simulink model "Sample_task"  (Simulink 8.1)
settings: Solver=ode4  SolverMode=SingleTasking  StartTime=0.0  StopTime=inf  FixedStep=0.0005  RelTol=1e-3
model workspace (MAT data in the model file):
  BKIN_STEP_TIME = 0.0005
  col_x = 1
  col_y = 2
  WIDTH = 3
  HEIGHT = 4
  TARGET_COL = 1
  LOAD = 2
  TRAJ_DURATION_COL = 3
  MAX_LOAD = 2
  FORCE_ON = 1
  HAND_RADIUS = 6
  REST_COL = 4
  TRAINING_COL = 5
  HAND_COLOR = 5
  TARGET_STROKE = 8
  TARGET_RADIUS = 9
  xMaxCursor = 15
  yMaxCursor = 16
  TARGET_COLOR = 7
  START_X = 10
  START_Y = 11
  END_X = 12
  END_Y = 13
  OPACITY_GRADIENT : num (value not decoded)
StartFcn:
  |  warndlg('Dexterit-E models cannot run under simulation. Please compile your model and run it from within Dexterit-E.');set_param(bdroot,'SimulationCommand','stop')
undefined symbols (not defined in the file or in its folder): slselsubs
libraries: simulink x4, General x3, KINARM_loads x2, KINARM_IO x1, KINARM_EP_loads x1, Video x1, xpclib x1
(part 1 of 3)
CloseFcn:
  | rtwprivate ssgencode ModelCloseRequest b2lab2d
settings Model: Creator=Chris Grebeldinger  LastModifiedBy=BKIN TECHNOLOGIES  ModifiedComment=chris -- Wed Feb 16 09:18:30 2005 -- Version 1.1384  ModifiedHistory=Feb 16/05 - Add error repeat, add offset ramp  ExtModeArmWhenConnect=off  ExtModeLogAll=off  BufferReuse=off
settings DataIOCC: LimitDataPoints=off  SaveOutput=off  SaveTime=off  SignalLoggingName=sigsOut
settings OptimizationCC: BlockReduction=off  BooleanDataType=off  OptimizeBlockIOStorage=off  BufferReuse=off  ExpressionFolding=off  FoldNonRolledExpr=off  LocalBlockOutputs=off  InitFltsAndDblsToZero=on
settings DebuggingCC: SaveWithParameterizedLinksMsg=none  SignalResolutionControl=TryResolveAllWithWarning  SolverPrmCheckMsg=none  MultiTaskDSMMsg=warning  MultiTaskCondExecSysMsg=none  StrictBusMsg=None
settings HardwareCC: ProdIntDivRoundTo=Zero  ProdEndianess=LittleEndian  ProdHWDeviceType=Generic->32-bit x86 compatible  TargetHWDeviceType=32-bit Generic
settings SFSimCC: SimParseCustomCode=off
settings RTWCC: SystemTargetFile=xpctarget.tlc  TemplateMakefile=xpc_default_tmf  Description=xPC Target  ProcessScript=xpctarget_make_rtw_hook  IncludeERTFirstTime=on  RTWCompilerOptimization=On
settings CodeAppCC: MaxIdLength=63
settings xpcTargetCC: TargetFcnLib=ansi_tfl_tmw.mat  CodeReplacementLibrary=XPC_BLAS  ParMdlRefBuildCompliant=on  ConcurrentExecutionCompliant=on  CombineSignalStateStructs=off  MATLABClassNameForMDSCustomization=xpcAperiodicCustomization  GRTInterface=on  GenerateAllocFcn=off  xPCTaskExecutionProfile=off  xPCRL32EventNumber=5000  xPCisDownloadable=off  xPCLoadParamSetFile=off  xPCConcurrentTasks=off  xPCEnableSFAnimation=off

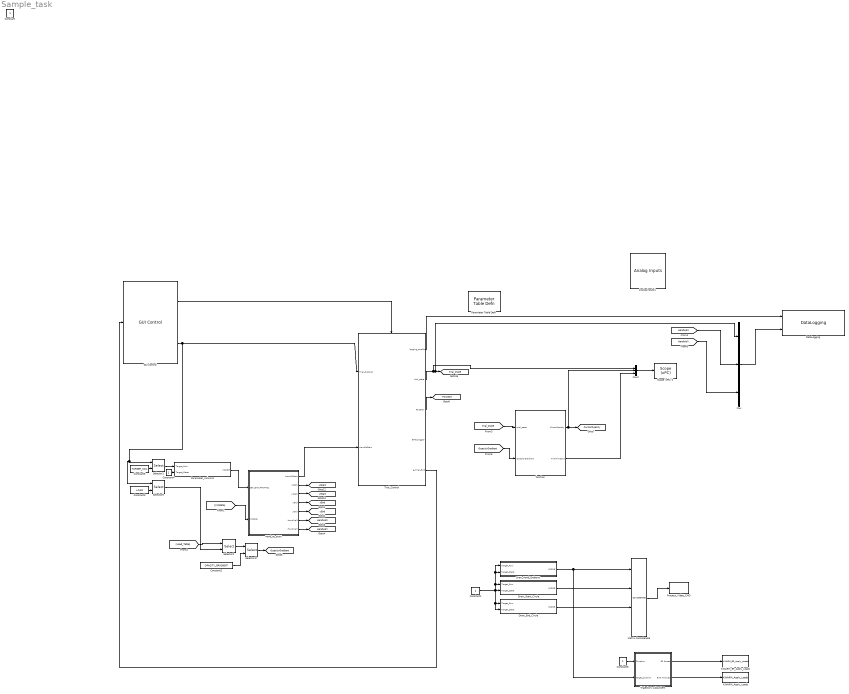
== system Sample_task ==
  Analog Inputs1 : KINARM_IO/Analog Inputs  channel=[5,6,7,8,9,10]  range=[5]  coupling=[0]  scantime6071e=1.28e-5  scantime6229=5e-6  sampletime=0.001  slot=-1  oscantime6071e=0
  Constant1 : Constant
  Constant2 : Constant  Value=OPACITY_GRADIENT
  Constant3 : Constant  Value=LOAD
  Constant4 : Constant
  Constant5 : Constant  Value=TARGET_COL
  Constant6 : Constant
  DataLogging : General/DataLogging  log_event_codes=off  log_analog_inputs=on
      link override Poll KINARM/EPTorqueCMD: GotoTag=KINARMEPTorqueCMD
      link override Poll KINARM/TorqueCMD: GotoTag=KINARMTorqueCMD
      link override Poll KINARM/ZeroEPTorque: Value=[0 0 0 0]
      link override Poll KINARM/ZeroTorque: Value=[0 0 0 0]
  Draw_End_Circle : Subsystem  AncestorBlock=Video/Show_Target_With_Label  mask(Show_Target_With_Label){target_type=Circle, num_states=1, attribcol1=[TARGET_COLOR TARGET_COLOR TARGET_STROKE TARGET_RADIUS 0 0 0], attribcol2=[6 6 0 3 0 0 0], attribcol3=[0 0 0 0 0 0 0], attribcol4=[0 0 0 0 0 0 0], attribcol5=[0 0 24 0 0 0 0], stateindices_padding=[0 0 0 0;0 0 0 0;0 0 0 0;0 0 0 0;0 0 0 0], source=dialog, opacity=100, target_display=Both subject and operator displays}
      mask prompts: target_type "Type of Target"; num_states "Number of Target States"; attribcol1 "State 1 Target Table Column(s)"; attribcol2 "State 2 Target Table Column(s)"; attribcol3 "State 3 Target Table Column(s)"; attribcol4 "State 4 Target Table Column(s)"; attribcol5 "State 5 Target Table Column(s)"; stateindices_padding "State Indices Padding"; source "Source for Opacity"; target_display "Target Display"
      mask help: This block returns a VCODE that, when sent to the Process_Video_CMD block, will cause a single target with a text label to be drawn. The label will be centered at the centroid of the target. Target parameters are specified in the Target Table according to the columns defined below and the row input to this block.
      mask init:
      | block_path = gcb;  % store block path, as gcb may change with block operations
      | 
      | %%% Get the model's workspace, because it is required to evaluate constants from the Parameter Table Def'n block
      | modelName=bdroot(block_path);
      | modelWorkspace = get_param(modelName, 'ModelWorkspace');
      | 
      | %%% Handle background colours if link status changes.  
      | checkBackgroundColour(block_path, 'Video');
      | 
      | %%% create the names of the input and output ports to display on the mask
      | output_block=char(find_system(block_path,'LookUnderMasks','all','FollowLinks','on','SearchDepth',1,'BlockType','Outport'));
      | outputname=get_param(output_block,'Name');
      | 
      | input_block=find_system(block_path,'LookUnderMasks','all','FollowLinks','on','SearchDepth',1,'BlockType','Inport');
      | inputname1=get_param(char(input_block{1}),'Name');
      | inputname2=get_param(char(input_block{2}),'Name');
      | if length(input_block) >= 3
      |     inputname3=get_param(char(input_block{3}),'Name');
      | end
      | 
      | %%%%%%%%%%%%%%%%%%%%%%%%%%%%%%%%%%%%%%%%%%%%%%%%%%%%%%%%%%%%%
      | %%% Create or replace the opacity input port
      | % Note: in earlier versions of MATLAB, the replace_block function did not work properly. When we drop support for R2007b,
      | % Check to see if it works properly in R2010a and if so, then this code can be simplified with the use of the replace_block function
      | sourceStr=get_param(block_path,'source');
      | 
      | if strmatch(sourceStr, 'dialog')
      | 	if length(input_block) == 3
      | 		pos=get_param([block_path '/Opacity'],'position');
      | 		delete_line(block_path, 'Opacity/1', 'Embedded MATLAB Function/4');
      | 		delete_block(input_block{3});
      |         add_block('built-in/Constant',[block_path '/Opacity'],'Name','Opacity');
      | 		set_param([block_path '/Opacity'],'position',pos);
      | 		add_line(block_path, 'Opacity/1', 'Embedded MATLAB Function/4');
      | 		set_param([block_path '/Opacity'],'Value','opacity');
      | 	end
      | 	displaytext = ['disp(columntext); port_label(''output'',1,outputname); port_label(''input'',1, inputname1); port_label(''input'',2, inputname2);'];
      | else
      | 	if length(input_block) == 2
      | 		pos=get_param([block_path '/Opacity'],'position');
      | 		delete_line(block_path, 'Opacity/1', 'Embedded MATLAB Function/4');
      | 		delete_block([block_path, '/Opacity']);
      | 		add_block('built-in/Inport',[block_path '/In2'],'Name','Opacity');
      | 		set_param([block_path '/Opacity'],'position',pos);
      | 		add_line(block_path, 'Opacity/1', 'Embedded MATLAB Function/4');
      |  	end
      | 	inputname3='Opacity';
      | 	displaytext = ['disp(columntext); port_label(''output'',1,outputname); port_label(''input'',1, inputname1); port_label(''input'',2, inputname2); port_label(''input'',3, inputname3);'];
      | end
      | set_param(block_path,'MaskDisplay',displaytext);
      | 
      | 
      | %%%%%%%%%%%%%%%%%%%%%%%%%%%%%%%%%%%%%%%%%%%%%%%%%%%%%%%%%%%%%
      | %%% Check and format the input strings for the vectors of column entires
      | targetTypeStr=get_param(block_path, 'target_type');
      | 
      | switch targetTypeStr(1:3)
      | 	case 'Cir',		numCol = 7;
      | 	case 'Ell',		numCol = 9;
      |     case 'Rec',		numCol = 9;
      |     case 'Lin',		numCol = 8;
      |     case 'Tri',		numCol = 10;
      | 	otherwise,		numCol = 7;
      | end
      | 
      | % % % numCol=str2num( get_param(block_path, 'num_col') );
      | for ii = 1:5
      | 	variableName = ['attribcol' num2str(ii)];
      | 	attribcoltext = get_param(block_path, variableName);
      | 	attribcoltext = checkUserInputVectorLength(attribcoltext, numCol);
      | 	set_param(block_path, variableName, attribcoltext);
      | end
      | 
      | % the input to the Embedded MATLAB script under the mask needs to have a certain size. This creates 'padding' to add to the 
      | % attribcol vectors to get to that size
      | zeros_5x7_matrix = zeros(5,7);
      | set_param(block_path, 'stateindices_padding', mat2str(zeros_5x7_matrix(:, 1:(11-numCol))) );
      | 
      | 
      | %%%%%%%%%%%%%%%%%%%%%%%%%%%%%%%%%%%%%%%%%%%%%%%%%%%%%%%%%%%%%
      | %%% Create the text to show on the mask
      | numStates = str2num(get_param(block_path, 'num_states'));
      | 
      | for ii = 1:numStates
      | 	variableName = ['attribcol' num2str(ii)];
      | 	attribcolString = get_param(block_path, variableName);
      | 	if isempty(modelWorkspace)
      | 		% if the block is part of a library, then modelWorkspace will be empty and the other code to evaluate attribcolStringEval will fail
      | 		attribcolStringEval = '[4 0 3 0 0 0 0]';
      | 	else
      | 		[attribcolValue, errorMessage] = BKINevalin(modelWorkspace, attribcolString);
      | 		attribcolStringEval = ['          ' mat2str( attribcolValue )];
      | 	end
      | 	if ii > 1
      | 		columntext = strvcat(columntext, attribcolStringEval);
      | 	else
      | 		columntext = attribcolStringEval;
      | 	end
      | end
      | 
      | % Add formatting spaces so that the mask looks nice
      | space = repmat(' ', 1, round(length(columntext)/2));
      | columntext=strvcat([space '(columns)'], columntext);
      mask Help:
      | Used to draw a single, stationary target with a label.
      | 
      | <H2>Library </H2>
      | Video
      | 
      | <H2>Description </H2>
      | This block returns a VCODE, which when sent to the Process_Video_CMD block will draw a single stationary target with a label. The VCODE contains all of the target parameters necessary to draw the target and the label.
      | <P>
      | The VCODE is generated from information contained in the Target Table. Which parts of the Target Table are used is determined by the columns selected (see Parameters and Dialog Box below).<P>
      | 
      | <p>For example, assume the "row" input is 2, the "type of target" is set to "rectangle" and the "Target Table Columns" is set to [3 0 0 4 5 0 6 7 4].
      | Then using the sample target table below a red rectangle will be drawn at (20cm, 40cm) with a width of 10cm and a height of 3cm.
      | The rectangle will have the word "Maybe" in yellow on it in letters 3cm heigh. The zeros in the  "Target Table Columns" indicate those parameters are not used (i.e. no stroke color, no stroke width, and no rotation).
      | 
      | <p><tt>
      | ______________________________________________________________________<br>
      | |&nbsp;&nbsp;&nbsp;&nbsp;&nbsp;&nbsp;&nbsp;&nbsp;&nbsp;&nbsp;| X Pos | Y pos |&nbsp;&nbsp;Fill | Width | Height |&nbsp;&nbsp;Text | TColor |<br>
      | ----------------------------------------------------------------------<br>
      | | target 1 |&nbsp;&nbsp;&nbsp;&nbsp;10 |&nbsp;&nbsp;&nbsp;&nbsp;10 | white |&nbsp;&nbsp;&nbsp;&nbsp;&nbsp;5 |&nbsp;&nbsp;&nbsp;&nbsp;&nbsp;&nbsp;2 |&nbsp;&nbsp;&nbsp;Yes |&nbsp;&nbsp;green |<br>
      | | target 2 |&nbsp;&nbsp;&nbsp;&nbsp;20 |&nbsp;&nbsp;&nbsp;&nbsp;40 |&nbsp;&nbsp;&nbsp;red |&nbsp;&nbsp;&nbsp;&nbsp;10 |&nbsp;&nbsp;&nbsp;&nbsp;&nbsp;&nbsp;3 | Maybe | yellow |<br>
      | | target 3 |&nbsp;&nbsp;&nbsp;-40 |&nbsp;&nbsp;&nbsp;&nbsp;10 |&nbsp;&nbsp;blue |&nbsp;&nbsp;&nbsp;&nbsp;&nbsp;3 |&nbsp;&nbsp;&nbsp;&nbsp;&nbsp;&nbsp;4 | Wrong |&nbsp;&nbsp;&nbsp;&nbsp;red |
      | ----------------------------------------------------------------------<br>
      | 
      | 
      | </tt>
      | 
      | 
      | <p>Inputs:<br>
      | <B> Target_Row: </B> this scalar input determines which row in the Target Table is used to define the target parameters. Typically the Target_Row comes from the Trial_Protocol.  <P>
      | <B> Target_State: </B> this scalar input determines which state the target is in. Different states reference different columns in the Target Table (as defined in the Dialog Box). Typically the Target_State input is controlled by the Stateflow chart to dynamically change the appearance of the target depending on system and/or subject behavior. Target_State=0 is a valid input, which turns the target off. The intended method for turning a target off is to set Target_State=0. <BR>
      | <P>
      | <B>Opacity:</B> This input is only available if Source for Opacity is selected as port, in which case the opacity for all of the targets created by this block is specified as a percentage.
      | The length of this input must either match the length of the Target_Row(s) input (i.e. which case each Opacity maps to the appropriate Target_row)
      | or this input must be a scalar (in which case the Opacity maps to all of the Target_Rows).<BR>
      | <P>
      | There is one output from this block:
      | <P>
      | <B> VCODE: </B> this output is a vector containing one VCODE. This output must go to the Process_Video_CMD block of the video library for the target to actually be shown (if any other visual targets are to be displayed, then this VCODE output must be concatenated with the other VCODES prior to connection to the Process_Video_CMD block - see Help for the Process_Video_CMD block for more information).
      | <P>
      | To show multiple targets simultaneously, multiple copies of the Show_Target and Show_Target_With_Label blocks can be used in a Task Program. The output VCODES from multiple Show_Target and Show_Target_With_Label blocks must be concatenated prior to connection to the Process_Video_CMD block.
      | <P>
      | 
      | <H2>Parameters and Dialog Box</H2>
      | <B>Type of Target:</B> Choose the type of target specified in the target table.
      | <P>
      | <B>Number of Target States:</B> Choose the number of target states specified in each target row. Up to five target states are allowed per target row.
      | <P>
      | <B>State [n] Target Table Columns:</B> Enter the column indices that specify the relevant target attributes in the Target Table. All target types have the same first three target attributes (fill colour, stroke colour and stroke width) and the same last three target attributes (label text, label colour, and label height).
      | <Blockquote>
      | <P>
      | Element 1 (fill colour) - points to the column index in the Target Table containing the fill colour. If this index is 0, then the fill colour is transparent and the Target Table is not referenced. For line targets, the fill colour is not used.
      | <P>
      | Element 2 (stroke colour) - points to the column index in the Target Table containing the stroke colour. If this index is 0, then the stroke colour is transparent and the Target Table is not referenced. It is possible to use the same column index for both fill colour and stroke colour (i.e.  if single-colour targets are desired). For line targets, stroke colour defines the colour of the line.
      | <P>
      | Element 3 (stroke width) - points to the column index in the Target Table containing the stroke width (cm). If no stroke is desired, then setting the stroke column index to 0 will produce a stroke width of 0  and the Target Table is not referenced.  Setting stroke column index to a value less than 0 will produce a standard 1 mm stroke width, again without referencing the Target Table. For line targets, stroke width defines the width of the line.
      | <P>
      | <B><I>Circle</I></B> <P>
      | Element 4 (radius) - radius of the circle (cm).
      | <P>
      | <B><I>Ellipse</I></B> <P>
      | Elements 4-6 (ellipse properties) - major radius (cm), minor radius (cm), rotation angle (degrees). If no rotation is desired, then setting rotation column index to 0 will produce a default rotation of 0 and the Target Table will not be referenced.
      | <P>
      | <B><I>Rectangle</I></B><P>
      | Elements 4-6 (rectangle properties) - length (cm), height (cm), rotation angle (degrees). If no rotation is desired, then setting rotation column index to 0 will produce a default rotation of 0 and the Target Table will not be referenced.
      | <P>
      | <B><I>Line</I></B><P>
      | Elements 4-5 (line properties) - end point x-axis position relative to start point (cm), end point y-axis position relative to start point (cm). The width and colour of the line are defined by the stroke width and the stroke colour, respectively. The fill colour column is ignored (i.e. any value can be used for column 1)
      | <P>
      | <B><I>Triangle</I></B><P>
      | Elements 4-7 (triangle properties) - length (cm), height (cm), offset of peak of triangle relative to midpoint of the length (cm), rotation angle (degrees). If a height column index of 0 is specified, then an equilateral triangle with sides of the specified length will be created and the Target Table will not be referenced for height or peak offset. If no rotation is desired, then setting a rotation column index of 0 will produce a default rotation of 0 and the Target Table will not be referenced.
      | <P>
      | <B><I>Label</I></B>
      | <P>
      | The last three elements of the target state vector define the label. In order, these elements are:
      | <P>
      | Label text - the index of the column in the Target Table containing the text used for the label (up to 50 characters).
      | <P>
      | Label colour - the index of the column in the Target Table containing the label colour. If this index is 0, then the label colour is transparent and the Target Table is not referenced.
      | <P>
      | Label height - the index of the column in the Target Table containing the label height (cm).
      | </Blockquote>
      | <P>
      | Each target state requires its own set of column index definitions (although multiple states can point to the same column index if desired).<P>
      | 
      | <B>Source for Opacity:</B> Choose either dialog, to specify the opacity in this dialog, or port, which will create a new input to allow dynamic control of opacity.
      | <P>
      | <B>Opacity:</B> This parameter is only available if Source for Opacity is selected as dialog, in which case the opacity for all of the targets created by this block is specified as a percentage.
      | <P>
      | <B>Target Display:</B> This option determines whether the target(s) are shown on the operator display only, the subject display only, or both displays.
      | <P>
      | 
      | <H2>Examples</H2>
      | 
      | <B>Example 1:</B>  Suppose a target row will be used to define 1 state for an ellipse type target. It will be an outline of an ellipse with a label in the center (using a stroke colour and a standard 1mm stroke width). The related Target Table columns are:
      | <P>
      | column 4 = colour<BR>
      | column 5 = major radius<BR>
      | column 6 = minor radius<BR>
      | column 7 = orientation<BR>
      | column 8 = label text<BR>
      | column 9 = label colour<BR>
      | column 10 = label height
      | <P>For this example, "State 1 Target Table Columns" would equal [0 4 -1 5 6 7 8 9 10].
      | <P>
      | 
      | <H2>Related Blocks </H2>
      | Show_Target<BR>
      | Process_Video_CMD
      mask TypeOptions target_type: Circle | Ellipse | Rectangle | Line | Triangle
      mask Callback target_type:
      | %%%%
      | % Because of bugs iN R2007, R2010a and R2013a (which have been reported to Mathworks), the following code
      | % is required here because in the Initialization Section it will ONLY correctly update those Mask Parameters that are hidden
      | % when the OK button is clicked (NOTE: the initialization code will correctly update all Mask Parameters when the Apply button
      | % is clicked, the bug is that it should also update everything when the OK button is clicked in the absence of an Apply click)
      | %
      | % Adding a set_param call which updates one of the mask parameters will call the initialization code to run, which "avoids"
      | % this bug. This code should be removed once Mathworks has fixed this bug.
      | 
      | temp = get_param(gcb, 'target_type');
      | set_param(gcb, 'target_type', temp);
      mask TypeOptions num_states: 1 | 2 | 3 | 4 | 5
      mask Callback num_states:
      | block_path=gcb;
      | num_states=str2num(get_param(block_path, 'num_states'));
      | vis=get_param(block_path,'MaskVisibilities');
      | 
      | %If the number of states>1, then output an array instead of a vector.
      | %Only show those inputs necessary on the Mask
      | output_block=char(find_system(block_path,'LookUnderMasks','all','SearchDepth',1,'BlockType','Outport'));
      | if num_states==1			%output of HandInTarget block is a vector
      | 	vis{4}='off';
      | 	vis{5}='off';
      | 	vis{6}='off';
      | 	vis{7}='off';
      | elseif num_states==2					%output of HandInTarget block is an array
      | 	vis{4}='on';
      | 	vis{5}='off';
      | 	vis{6}='off';
      | 	vis{7}='off';
      | elseif num_states==3					%output of HandInTarget block is an array
      | 	vis{4}='on';
      | 	vis{5}='on';
      | 	vis{6}='off';
      | 	vis{7}='off';
      | elseif num_states==4					%output of HandInTarget block is an array
      | 	vis{4}='on';
      | 	vis{5}='on';
      | 	vis{6}='on';
      | 	vis{7}='off';
      | else								%output of HandInTarget block is an array
      | 	vis{4}='on';
      | 	vis{5}='on';
      | 	vis{6}='on';
      | 	vis{7}='on';
      | end
      | set_param(block_path,'MaskVisibilities',vis);
      mask TypeOptions source: dialog | port
      mask Callback source:
      | % Show or hide the opacity input on the mask dialog
      | sourceStr=get_param(gcb,'source');
      | vis=get_param(gcb,'MaskVisibilities');
      | 
      | if strmatch(sourceStr, 'dialog')
      | 	vis{10}='on';
      | else
      | 	vis{10}='off';
      | end
      | 
      | set_param(gcb,'MaskVisibilities',vis);
      mask TypeOptions target_display: Both subject and operator displays | Subject display only | Operator display only
      mask Display: disp(columntext); port_label('output',1,outputname); port_label('input',1, inputname1); port_label('input',2, inputname2);
  Draw_Hand_Endpoint : Subsystem  AncestorBlock=Video/Show_Target_With_Label  mask(Show_Target_With_Label){target_type=Circle, num_states=1, attribcol1=[HAND_COLOR 0 0 HAND_RADIUS 0 0 0], attribcol2=[6 6 0 3 0 0 0], attribcol3=[0 0 0 0 0 0 0], attribcol4=[0 0 0 0 0 0 0], attribcol5=[0 0 24 0 0 0 0], stateindices_padding=[0 0 0 0;0 0 0 0;0 0 0 0;0 0 0 0;0 0 0 0], source=dialog, opacity=100, target_display=Both subject and operator displays}
      mask prompts: target_type "Type of Target"; num_states "Number of Target States"; attribcol1 "State 1 Target Table Column(s)"; attribcol2 "State 2 Target Table Column(s)"; attribcol3 "State 3 Target Table Column(s)"; attribcol4 "State 4 Target Table Column(s)"; attribcol5 "State 5 Target Table Column(s)"; stateindices_padding "State Indices Padding"; source "Source for Opacity"; target_display "Target Display"
      mask help: This block returns a VCODE that, when sent to the Process_Video_CMD block, will cause a single target with a text label to be drawn. The label will be centered at the centroid of the target. Target parameters are specified in the Target Table according to the columns defined below and the row input to this block.
      mask init: same as Sample_task/Draw_End_Circle
      mask Help:
      | Used to draw a single, stationary target with a label.
      | 
      | <H2>Library </H2>
      | Video
      | 
      | <H2>Description </H2>
      | This block returns a VCODE, which when sent to the Process_Video_CMD block will draw a single stationary target with a label. The VCODE contains all of the target parameters necessary to draw the target and the label.
      | <P>
      | The VCODE is generated from information contained in the Target Table. Which parts of the Target Table are used is determined by the columns selected (see Parameters and Dialog Box below).<P>
      | 
      | <p>For example, assume the "row" input is 2, the "type of target" is set to "rectangle" and the "Target Table Columns" is set to [3 0 0 4 5 0 6 7 4].
      | Then using the sample target table below a red rectangle will be drawn at (20cm, 40cm) with a width of 10cm and a height of 3cm.
      | The rectangle will have the word "Maybe" in yellow on it in letters 3cm heigh. The zeros in the  "Target Table Columns" indicate those parameters are not used (i.e. no stroke color, no stroke width, and no rotation).
      | 
      | <p><tt>
      | ______________________________________________________________________<br>
      | |&nbsp;&nbsp;&nbsp;&nbsp;&nbsp;&nbsp;&nbsp;&nbsp;&nbsp;&nbsp;| X Pos | Y pos |&nbsp;&nbsp;Fill | Width | Height |&nbsp;&nbsp;Text | TColor |<br>
      | ----------------------------------------------------------------------<br>
      | | target 1 |&nbsp;&nbsp;&nbsp;&nbsp;10 |&nbsp;&nbsp;&nbsp;&nbsp;10 | white |&nbsp;&nbsp;&nbsp;&nbsp;&nbsp;5 |&nbsp;&nbsp;&nbsp;&nbsp;&nbsp;&nbsp;2 |&nbsp;&nbsp;&nbsp;Yes |&nbsp;&nbsp;green |<br>
      | | target 2 |&nbsp;&nbsp;&nbsp;&nbsp;20 |&nbsp;&nbsp;&nbsp;&nbsp;40 |&nbsp;&nbsp;&nbsp;red |&nbsp;&nbsp;&nbsp;&nbsp;10 |&nbsp;&nbsp;&nbsp;&nbsp;&nbsp;&nbsp;3 | Maybe | yellow |<br>
      | | target 3 |&nbsp;&nbsp;&nbsp;-40 |&nbsp;&nbsp;&nbsp;&nbsp;10 |&nbsp;&nbsp;blue |&nbsp;&nbsp;&nbsp;&nbsp;&nbsp;3 |&nbsp;&nbsp;&nbsp;&nbsp;&nbsp;&nbsp;4 | Wrong |&nbsp;&nbsp;&nbsp;&nbsp;red |
      | ----------------------------------------------------------------------<br>
      | 
      | 
      | </tt>
      | 
      | 
      | <p>Inputs:<br>
      | <B> Target_Row: </B> this scalar input determines which row in the Target Table is used to define the target parameters. Typically the Target_Row comes from the Trial_Protocol.  <P>
      | <B> Target_State: </B> this scalar input determines which state the target is in. Different states reference different columns in the Target Table (as defined in the Dialog Box). Typically the Target_State input is controlled by the Stateflow chart to dynamically change the appearance of the target depending on system and/or subject behavior. Target_State=0 is a valid input, which turns the target off. The intended method for turning a target off is to set Target_State=0. <BR>
      | <P>
      | <B>Opacity:</B> This input is only available if Source for Opacity is selected as port, in which case the opacity for all of the targets created by this block is specified as a percentage.
      | The length of this input must either match the length of the Target_Row(s) input (i.e. which case each Opacity maps to the appropriate Target_row)
      | or this input must be a scalar (in which case the Opacity maps to all of the Target_Rows).<BR>
      | <P>
      | There is one output from this block:
      | <P>
      | <B> VCODE: </B> this output is a vector containing one VCODE. This output must go to the Process_Video_CMD block of the video library for the target to actually be shown (if any other visual targets are to be displayed, then this VCODE output must be concatenated with the other VCODES prior to connection to the Process_Video_CMD block - see Help for the Process_Video_CMD block for more information).
      | <P>
      | To show multiple targets simultaneously, multiple copies of the Show_Target and Show_Target_With_Label blocks can be used in a Task Program. The output VCODES from multiple Show_Target and Show_Target_With_Label blocks must be concatenated prior to connection to the Process_Video_CMD block.
      | <P>
      | 
      | <H2>Parameters and Dialog Box</H2>
      | <B>Type of Target:</B> Choose the type of target specified in the target table.
      | <P>
      | <B>Number of Target States:</B> Choose the number of target states specified in each target row. Up to five target states are allowed per target row.
      | <P>
      | <B>State [n] Target Table Columns:</B> Enter the column indices that specify the relevant target attributes in the Target Table. All target types have the same first three target attributes (fill colour, stroke colour and stroke width) and the same last three target attributes (label text, label colour, and label height).
      | <Blockquote>
      | <P>
      | Element 1 (fill colour) - points to the column index in the Target Table containing the fill colour. If this index is 0, then the fill colour is transparent and the Target Table is not referenced. For line targets, the fill colour is not used.
      | <P>
      | Element 2 (stroke colour) - points to the column index in the Target Table containing the stroke colour. If this index is 0, then the stroke colour is transparent and the Target Table is not referenced. It is possible to use the same column index for both fill colour and stroke colour (i.e.  if single-colour targets are desired). For line targets, stroke colour defines the colour of the line.
      | <P>
      | Element 3 (stroke width) - points to the column index in the Target Table containing the stroke width (cm). If no stroke is desired, then setting the stroke column index to 0 will produce a stroke width of 0  and the Target Table is not referenced.  Setting stroke column index to a value less than 0 will produce a standard 1 mm stroke width, again without referencing the Target Table. For line targets, stroke width defines the width of the line.
      | <P>
      | <B><I>Circle</I></B> <P>
      | Element 4 (radius) - radius of the circle (cm).
      | <P>
      | <B><I>Ellipse</I></B> <P>
      | Elements 4-6 (ellipse properties) - major radius (cm), minor radius (cm), rotation angle (degrees). If no rotation is desired, then setting rotation column index to 0 will produce a default rotation of 0 and the Target Table will not be referenced.
      | <P>
      | <B><I>Rectangle</I></B><P>
      | Elements 4-6 (rectangle properties) - length (cm), height (cm), rotation angle (degrees). If no rotation is desired, then setting rotation column index to 0 will produce a default rotation of 0 and the Target Table will not be referenced.
      | <P>
      | <B><I>Line</I></B><P>
      | Elements 4-5 (line properties) - end point x-axis position relative to start point (cm), end point y-axis position relative to start point (cm). The width and colour of the line are defined by the stroke width and the stroke colour, respectively. The fill colour column is ignored (i.e. any value can be used for column 1)
      | <P>
      | <B><I>Triangle</I></B><P>
      | Elements 4-7 (triangle properties) - length (cm), height (cm), offset of peak of triangle relative to midpoint of the length (cm), rotation angle (degrees). If a height column index of 0 is specified, then an equilateral triangle with sides of the specified length will be created and the Target Table will not be referenced for height or peak offset. If no rotation is desired, then setting a rotation column index of 0 will produce a default rotation of 0 and the Target Table will not be referenced.
      | <P>
      | <B><I>Label</I></B>
      | <P>
      | The last three elements of the target state vector define the label. In order, these elements are:
      | <P>
      | Label text - the index of the column in the Target Table containing the text used for the label (up to 50 characters).
      | <P>
      | Label colour - the index of the column in the Target Table containing the label colour. If this index is 0, then the label colour is transparent and the Target Table is not referenced.
      | <P>
      | Label height - the index of the column in the Target Table containing the label height (cm).
      | </Blockquote>
      | <P>
      | Each target state requires its own set of column index definitions (although multiple states can point to the same column index if desired).<P>
      | 
      | <B>Source for Opacity:</B> Choose either dialog, to specify the opacity in this dialog, or port, which will create a new input to allow dynamic control of opacity.
      | <P>
      | <B>Opacity:</B> This parameter is only available if Source for Opacity is selected as dialog, in which case the opacity for all of the targets created by this block is specified as a percentage.
      | <P>
      | <B>Target Display:</B> This option determines whether the target(s) are shown on the operator display only, the subject display only, or both displays.
      | <P>
      | 
      | <H2>Examples</H2>
      | 
      | <B>Example 1:</B>  Suppose a target row will be used to define 1 state for an ellipse type target. It will be an outline of an ellipse with a label in the center (using a stroke colour and a standard 1mm stroke width). The related Target Table columns are:
      | <P>
      | column 4 = colour<BR>
      | column 5 = major radius<BR>
      | column 6 = minor radius<BR>
      | column 7 = orientation<BR>
      | column 8 = label text<BR>
      | column 9 = label colour<BR>
      | column 10 = label height
      | <P>For this example, "State 1 Target Table Columns" would equal [0 4 -1 5 6 7 8 9 10].
      | <P>
      | 
      | <H2>Related Blocks </H2>
      | Show_Target<BR>
      | Process_Video_CMD
      mask TypeOptions target_type: Circle | Ellipse | Rectangle | Line | Triangle
      mask Callback target_type:
      | %%%%
      | % Because of bugs iN R2007, R2010a and R2013a (which have been reported to Mathworks), the following code
      | % is required here because in the Initialization Section it will ONLY correctly update those Mask Parameters that are hidden
      | % when the OK button is clicked (NOTE: the initialization code will correctly update all Mask Parameters when the Apply button
      | % is clicked, the bug is that it should also update everything when the OK button is clicked in the absence of an Apply click)
      | %
      | % Adding a set_param call which updates one of the mask parameters will call the initialization code to run, which "avoids"
      | % this bug. This code should be removed once Mathworks has fixed this bug.
      | 
      | temp = get_param(gcb, 'target_type');
      | set_param(gcb, 'target_type', temp);
      mask TypeOptions num_states: 1 | 2 | 3 | 4 | 5
      mask Callback num_states:
      | block_path=gcb;
      | num_states=str2num(get_param(block_path, 'num_states'));
      | vis=get_param(block_path,'MaskVisibilities');
      | 
      | %If the number of states>1, then output an array instead of a vector.
      | %Only show those inputs necessary on the Mask
      | output_block=char(find_system(block_path,'LookUnderMasks','all','SearchDepth',1,'BlockType','Outport'));
      | if num_states==1			%output of HandInTarget block is a vector
      | 	vis{4}='off';
      | 	vis{5}='off';
      | 	vis{6}='off';
      | 	vis{7}='off';
      | elseif num_states==2					%output of HandInTarget block is an array
      | 	vis{4}='on';
      | 	vis{5}='off';
      | 	vis{6}='off';
      | 	vis{7}='off';
      | elseif num_states==3					%output of HandInTarget block is an array
      | 	vis{4}='on';
      | 	vis{5}='on';
      | 	vis{6}='off';
      | 	vis{7}='off';
      | elseif num_states==4					%output of HandInTarget block is an array
      | 	vis{4}='on';
      | 	vis{5}='on';
      | 	vis{6}='on';
      | 	vis{7}='off';
      | else								%output of HandInTarget block is an array
      | 	vis{4}='on';
      | 	vis{5}='on';
      | 	vis{6}='on';
      | 	vis{7}='on';
      | end
      | set_param(block_path,'MaskVisibilities',vis);
      mask TypeOptions source: dialog | port
      mask Callback source:
      | % Show or hide the opacity input on the mask dialog
      | sourceStr=get_param(gcb,'source');
      | vis=get_param(gcb,'MaskVisibilities');
      | 
      | if strmatch(sourceStr, 'dialog')
      | 	vis{10}='on';
      | else
      | 	vis{10}='off';
      | end
      | 
      | set_param(gcb,'MaskVisibilities',vis);
      mask TypeOptions target_display: Both subject and operator displays | Subject display only | Operator display only
      mask Display: disp(columntext); port_label('output',1,outputname); port_label('input',1, inputname1); port_label('input',2, inputname2);
  Draw_Start_Circle : Subsystem  AncestorBlock=Video/Show_Target_With_Label  mask(Show_Target_With_Label){target_type=Circle, num_states=1, attribcol1=[TARGET_COLOR TARGET_COLOR TARGET_STROKE TARGET_RADIUS 0 0 0], attribcol2=[6 6 0 3 0 0 0], attribcol3=[0 0 0 0 0 0 0], attribcol4=[0 0 0 0 0 0 0], attribcol5=[0 0 24 0 0 0 0], stateindices_padding=[0 0 0 0;0 0 0 0;0 0 0 0;0 0 0 0;0 0 0 0], source=dialog, opacity=100, target_display=Both subject and operator displays}
      mask prompts: target_type "Type of Target"; num_states "Number of Target States"; attribcol1 "State 1 Target Table Column(s)"; attribcol2 "State 2 Target Table Column(s)"; attribcol3 "State 3 Target Table Column(s)"; attribcol4 "State 4 Target Table Column(s)"; attribcol5 "State 5 Target Table Column(s)"; stateindices_padding "State Indices Padding"; source "Source for Opacity"; target_display "Target Display"
      mask help: This block returns a VCODE that, when sent to the Process_Video_CMD block, will cause a single target with a text label to be drawn. The label will be centered at the centroid of the target. Target parameters are specified in the Target Table according to the columns defined below and the row input to this block.
      mask init: same as Sample_task/Draw_End_Circle
      mask Help:
      | Used to draw a single, stationary target with a label.
      | 
      | <H2>Library </H2>
      | Video
      | 
      | <H2>Description </H2>
      | This block returns a VCODE, which when sent to the Process_Video_CMD block will draw a single stationary target with a label. The VCODE contains all of the target parameters necessary to draw the target and the label.
      | <P>
      | The VCODE is generated from information contained in the Target Table. Which parts of the Target Table are used is determined by the columns selected (see Parameters and Dialog Box below).<P>
      | 
      | <p>For example, assume the "row" input is 2, the "type of target" is set to "rectangle" and the "Target Table Columns" is set to [3 0 0 4 5 0 6 7 4].
      | Then using the sample target table below a red rectangle will be drawn at (20cm, 40cm) with a width of 10cm and a height of 3cm.
      | The rectangle will have the word "Maybe" in yellow on it in letters 3cm heigh. The zeros in the  "Target Table Columns" indicate those parameters are not used (i.e. no stroke color, no stroke width, and no rotation).
      | 
      | <p><tt>
      | ______________________________________________________________________<br>
      | |&nbsp;&nbsp;&nbsp;&nbsp;&nbsp;&nbsp;&nbsp;&nbsp;&nbsp;&nbsp;| X Pos | Y pos |&nbsp;&nbsp;Fill | Width | Height |&nbsp;&nbsp;Text | TColor |<br>
      | ----------------------------------------------------------------------<br>
      | | target 1 |&nbsp;&nbsp;&nbsp;&nbsp;10 |&nbsp;&nbsp;&nbsp;&nbsp;10 | white |&nbsp;&nbsp;&nbsp;&nbsp;&nbsp;5 |&nbsp;&nbsp;&nbsp;&nbsp;&nbsp;&nbsp;2 |&nbsp;&nbsp;&nbsp;Yes |&nbsp;&nbsp;green |<br>
      | | target 2 |&nbsp;&nbsp;&nbsp;&nbsp;20 |&nbsp;&nbsp;&nbsp;&nbsp;40 |&nbsp;&nbsp;&nbsp;red |&nbsp;&nbsp;&nbsp;&nbsp;10 |&nbsp;&nbsp;&nbsp;&nbsp;&nbsp;&nbsp;3 | Maybe | yellow |<br>
      | | target 3 |&nbsp;&nbsp;&nbsp;-40 |&nbsp;&nbsp;&nbsp;&nbsp;10 |&nbsp;&nbsp;blue |&nbsp;&nbsp;&nbsp;&nbsp;&nbsp;3 |&nbsp;&nbsp;&nbsp;&nbsp;&nbsp;&nbsp;4 | Wrong |&nbsp;&nbsp;&nbsp;&nbsp;red |
      | ----------------------------------------------------------------------<br>
      | 
      | 
      | </tt>
      | 
      | 
      | <p>Inputs:<br>
      | <B> Target_Row: </B> this scalar input determines which row in the Target Table is used to define the target parameters. Typically the Target_Row comes from the Trial_Protocol.  <P>
      | <B> Target_State: </B> this scalar input determines which state the target is in. Different states reference different columns in the Target Table (as defined in the Dialog Box). Typically the Target_State input is controlled by the Stateflow chart to dynamically change the appearance of the target depending on system and/or subject behavior. Target_State=0 is a valid input, which turns the target off. The intended method for turning a target off is to set Target_State=0. <BR>
      | <P>
      | <B>Opacity:</B> This input is only available if Source for Opacity is selected as port, in which case the opacity for all of the targets created by this block is specified as a percentage.
      | The length of this input must either match the length of the Target_Row(s) input (i.e. which case each Opacity maps to the appropriate Target_row)
      | or this input must be a scalar (in which case the Opacity maps to all of the Target_Rows).<BR>
      | <P>
      | There is one output from this block:
      | <P>
      | <B> VCODE: </B> this output is a vector containing one VCODE. This output must go to the Process_Video_CMD block of the video library for the target to actually be shown (if any other visual targets are to be displayed, then this VCODE output must be concatenated with the other VCODES prior to connection to the Process_Video_CMD block - see Help for the Process_Video_CMD block for more information).
      | <P>
      | To show multiple targets simultaneously, multiple copies of the Show_Target and Show_Target_With_Label blocks can be used in a Task Program. The output VCODES from multiple Show_Target and Show_Target_With_Label blocks must be concatenated prior to connection to the Process_Video_CMD block.
      | <P>
      | 
      | <H2>Parameters and Dialog Box</H2>
      | <B>Type of Target:</B> Choose the type of target specified in the target table.
      | <P>
      | <B>Number of Target States:</B> Choose the number of target states specified in each target row. Up to five target states are allowed per target row.
      | <P>
      | <B>State [n] Target Table Columns:</B> Enter the column indices that specify the relevant target attributes in the Target Table. All target types have the same first three target attributes (fill colour, stroke colour and stroke width) and the same last three target attributes (label text, label colour, and label height).
      | <Blockquote>
      | <P>
      | Element 1 (fill colour) - points to the column index in the Target Table containing the fill colour. If this index is 0, then the fill colour is transparent and the Target Table is not referenced. For line targets, the fill colour is not used.
      | <P>
      | Element 2 (stroke colour) - points to the column index in the Target Table containing the stroke colour. If this index is 0, then the stroke colour is transparent and the Target Table is not referenced. It is possible to use the same column index for both fill colour and stroke colour (i.e.  if single-colour targets are desired). For line targets, stroke colour defines the colour of the line.
      | <P>
      | Element 3 (stroke width) - points to the column index in the Target Table containing the stroke width (cm). If no stroke is desired, then setting the stroke column index to 0 will produce a stroke width of 0  and the Target Table is not referenced.  Setting stroke column index to a value less than 0 will produce a standard 1 mm stroke width, again without referencing the Target Table. For line targets, stroke width defines the width of the line.
      | <P>
      | <B><I>Circle</I></B> <P>
      | Element 4 (radius) - radius of the circle (cm).
      | <P>
      | <B><I>Ellipse</I></B> <P>
      | Elements 4-6 (ellipse properties) - major radius (cm), minor radius (cm), rotation angle (degrees). If no rotation is desired, then setting rotation column index to 0 will produce a default rotation of 0 and the Target Table will not be referenced.
      | <P>
      | <B><I>Rectangle</I></B><P>
      | Elements 4-6 (rectangle properties) - length (cm), height (cm), rotation angle (degrees). If no rotation is desired, then setting rotation column index to 0 will produce a default rotation of 0 and the Target Table will not be referenced.
      | <P>
      | <B><I>Line</I></B><P>
      | Elements 4-5 (line properties) - end point x-axis position relative to start point (cm), end point y-axis position relative to start point (cm). The width and colour of the line are defined by the stroke width and the stroke colour, respectively. The fill colour column is ignored (i.e. any value can be used for column 1)
      | <P>
      | <B><I>Triangle</I></B><P>
      | Elements 4-7 (triangle properties) - length (cm), height (cm), offset of peak of triangle relative to midpoint of the length (cm), rotation angle (degrees). If a height column index of 0 is specified, then an equilateral triangle with sides of the specified length will be created and the Target Table will not be referenced for height or peak offset. If no rotation is desired, then setting a rotation column index of 0 will produce a default rotation of 0 and the Target Table will not be referenced.
      | <P>
      | <B><I>Label</I></B>
      | <P>
      | The last three elements of the target state vector define the label. In order, these elements are:
      | <P>
      | Label text - the index of the column in the Target Table containing the text used for the label (up to 50 characters).
      | <P>
      | Label colour - the index of the column in the Target Table containing the label colour. If this index is 0, then the label colour is transparent and the Target Table is not referenced.
      | <P>
      | Label height - the index of the column in the Target Table containing the label height (cm).
      | </Blockquote>
      | <P>
      | Each target state requires its own set of column index definitions (although multiple states can point to the same column index if desired).<P>
      | 
      | <B>Source for Opacity:</B> Choose either dialog, to specify the opacity in this dialog, or port, which will create a new input to allow dynamic control of opacity.
      | <P>
      | <B>Opacity:</B> This parameter is only available if Source for Opacity is selected as dialog, in which case the opacity for all of the targets created by this block is specified as a percentage.
      | <P>
      | <B>Target Display:</B> This option determines whether the target(s) are shown on the operator display only, the subject display only, or both displays.
      | <P>
      | 
      | <H2>Examples</H2>
      | 
      | <B>Example 1:</B>  Suppose a target row will be used to define 1 state for an ellipse type target. It will be an outline of an ellipse with a label in the center (using a stroke colour and a standard 1mm stroke width). The related Target Table columns are:
      | <P>
      | column 4 = colour<BR>
      | column 5 = major radius<BR>
      | column 6 = minor radius<BR>
      | column 7 = orientation<BR>
      | column 8 = label text<BR>
      | column 9 = label colour<BR>
      | column 10 = label height
      | <P>For this example, "State 1 Target Table Columns" would equal [0 4 -1 5 6 7 8 9 10].
      | <P>
      | 
      | <H2>Related Blocks </H2>
      | Show_Target<BR>
      | Process_Video_CMD
      mask TypeOptions target_type: Circle | Ellipse | Rectangle | Line | Triangle
      mask Callback target_type:
      | %%%%
      | % Because of bugs iN R2007, R2010a and R2013a (which have been reported to Mathworks), the following code
      | % is required here because in the Initialization Section it will ONLY correctly update those Mask Parameters that are hidden
      | % when the OK button is clicked (NOTE: the initialization code will correctly update all Mask Parameters when the Apply button
      | % is clicked, the bug is that it should also update everything when the OK button is clicked in the absence of an Apply click)
      | %
      | % Adding a set_param call which updates one of the mask parameters will call the initialization code to run, which "avoids"
      | % this bug. This code should be removed once Mathworks has fixed this bug.
      | 
      | temp = get_param(gcb, 'target_type');
      | set_param(gcb, 'target_type', temp);
      mask TypeOptions num_states: 1 | 2 | 3 | 4 | 5
      mask Callback num_states:
      | block_path=gcb;
      | num_states=str2num(get_param(block_path, 'num_states'));
      | vis=get_param(block_path,'MaskVisibilities');
      | 
      | %If the number of states>1, then output an array instead of a vector.
      | %Only show those inputs necessary on the Mask
      | output_block=char(find_system(block_path,'LookUnderMasks','all','SearchDepth',1,'BlockType','Outport'));
      | if num_states==1			%output of HandInTarget block is a vector
      | 	vis{4}='off';
      | 	vis{5}='off';
      | 	vis{6}='off';
      | 	vis{7}='off';
      | elseif num_states==2					%output of HandInTarget block is an array
      | 	vis{4}='on';
      | 	vis{5}='off';
      | 	vis{6}='off';
      | 	vis{7}='off';
      | elseif num_states==3					%output of HandInTarget block is an array
      | 	vis{4}='on';
      | 	vis{5}='on';
      | 	vis{6}='off';
      | 	vis{7}='off';
      | elseif num_states==4					%output of HandInTarget block is an array
      | 	vis{4}='on';
      | 	vis{5}='on';
      | 	vis{6}='on';
      | 	vis{7}='off';
      | else								%output of HandInTarget block is an array
      | 	vis{4}='on';
      | 	vis{5}='on';
      | 	vis{6}='on';
      | 	vis{7}='on';
      | end
      | set_param(block_path,'MaskVisibilities',vis);
      mask TypeOptions source: dialog | port
      mask Callback source:
      | % Show or hide the opacity input on the mask dialog
      | sourceStr=get_param(gcb,'source');
      | vis=get_param(gcb,'MaskVisibilities');
      | 
      | if strmatch(sourceStr, 'dialog')
      | 	vis{10}='on';
      | else
      | 	vis{10}='off';
      | end
      | 
      | set_param(gcb,'MaskVisibilities',vis);
      mask TypeOptions target_display: Both subject and operator displays | Subject display only | Operator display only
      mask Display: disp(columntext); port_label('output',1,outputname); port_label('input',1, inputname1); port_label('input',2, inputname2);
  GUI Control : General/GUI Control  target_type_str=Circle  Target_Type=1  XYcols=[1 2]  Vcols=3  Lcols=4  indices_padding=[0 0 0 0;0 0 0 0]  task_version=1.0  show_repeat_trial_flag=off
  Hand_at_start : MATLAB Function  TreatAsAtomicUnit=on
  KINARM_Apply_Loads : KINARM_loads/KINARM_Apply_Loads  up_duration=1500  down_duration=1500  max_torque=10
  KINARM_EP_Apply_Loads : KINARM_EP_loads/KINARM_EP_Apply_Loads  up_duration=1500  down_duration=1500  max_force=60
  Matrix Concatenate : Concatenate  NumInputs=4  Mode=Multidimensional array
  Mux : Mux  Inputs=3
  Mux2 : Mux  Inputs=3
  Parameter Table Defn : General/Parameter Table Defn  ShowInLibBrowser=0
  Parameter_columns : Subsystem  AncestorBlock=Video/Show_Target_With_Label  mask(Show_Target_With_Label){target_type=Circle, num_states=1, attribcol1=[START_X START_Y END_X END_Y TARGET_RADIUS 0 0], attribcol2=[6 6 0 3 0 0 0], attribcol3=[0 0 0 0 0 0 0], attribcol4=[0 0 0 0 0 0 0], attribcol5=[0 0 24 0 0 0 0], stateindices_padding=[0 0 0 0;0 0 0 0;0 0 0 0;0 0 0 0;0 0 0 0], source=dialog, opacity=100, target_display=Both subject and operator displays}
      mask prompts: target_type "Type of Target"; num_states "Number of Target States"; attribcol1 "State 1 Target Table Column(s)"; attribcol2 "State 2 Target Table Column(s)"; attribcol3 "State 3 Target Table Column(s)"; attribcol4 "State 4 Target Table Column(s)"; attribcol5 "State 5 Target Table Column(s)"; stateindices_padding "State Indices Padding"; source "Source for Opacity"; target_display "Target Display"
      mask help: This block returns a VCODE that, when sent to the Process_Video_CMD block, will cause a single target with a text label to be drawn. The label will be centered at the centroid of the target. Target parameters are specified in the Target Table according to the columns defined below and the row input to this block.
      mask init: same as Sample_task/Draw_End_Circle
      mask Help:
      | Used to draw a single, stationary target with a label.
      | 
      | <H2>Library </H2>
      | Video
      | 
      | <H2>Description </H2>
      | This block returns a VCODE, which when sent to the Process_Video_CMD block will draw a single stationary target with a label. The VCODE contains all of the target parameters necessary to draw the target and the label.
      | <P>
      | The VCODE is generated from information contained in the Target Table. Which parts of the Target Table are used is determined by the columns selected (see Parameters and Dialog Box below).<P>
      | 
      | <p>For example, assume the "row" input is 2, the "type of target" is set to "rectangle" and the "Target Table Columns" is set to [3 0 0 4 5 0 6 7 4].
      | Then using the sample target table below a red rectangle will be drawn at (20cm, 40cm) with a width of 10cm and a height of 3cm.
      | The rectangle will have the word "Maybe" in yellow on it in letters 3cm heigh. The zeros in the  "Target Table Columns" indicate those parameters are not used (i.e. no stroke color, no stroke width, and no rotation).
      | 
      | <p><tt>
      | ______________________________________________________________________<br>
      | |&nbsp;&nbsp;&nbsp;&nbsp;&nbsp;&nbsp;&nbsp;&nbsp;&nbsp;&nbsp;| X Pos | Y pos |&nbsp;&nbsp;Fill | Width | Height |&nbsp;&nbsp;Text | TColor |<br>
      | ----------------------------------------------------------------------<br>
      | | target 1 |&nbsp;&nbsp;&nbsp;&nbsp;10 |&nbsp;&nbsp;&nbsp;&nbsp;10 | white |&nbsp;&nbsp;&nbsp;&nbsp;&nbsp;5 |&nbsp;&nbsp;&nbsp;&nbsp;&nbsp;&nbsp;2 |&nbsp;&nbsp;&nbsp;Yes |&nbsp;&nbsp;green |<br>
      | | target 2 |&nbsp;&nbsp;&nbsp;&nbsp;20 |&nbsp;&nbsp;&nbsp;&nbsp;40 |&nbsp;&nbsp;&nbsp;red |&nbsp;&nbsp;&nbsp;&nbsp;10 |&nbsp;&nbsp;&nbsp;&nbsp;&nbsp;&nbsp;3 | Maybe | yellow |<br>
      | | target 3 |&nbsp;&nbsp;&nbsp;-40 |&nbsp;&nbsp;&nbsp;&nbsp;10 |&nbsp;&nbsp;blue |&nbsp;&nbsp;&nbsp;&nbsp;&nbsp;3 |&nbsp;&nbsp;&nbsp;&nbsp;&nbsp;&nbsp;4 | Wrong |&nbsp;&nbsp;&nbsp;&nbsp;red |
      | ----------------------------------------------------------------------<br>
      | 
      | 
      | </tt>
      | 
      | 
      | <p>Inputs:<br>
      | <B> Target_Row: </B> this scalar input determines which row in the Target Table is used to define the target parameters. Typically the Target_Row comes from the Trial_Protocol.  <P>
      | <B> Target_State: </B> this scalar input determines which state the target is in. Different states reference different columns in the Target Table (as defined in the Dialog Box). Typically the Target_State input is controlled by the Stateflow chart to dynamically change the appearance of the target depending on system and/or subject behavior. Target_State=0 is a valid input, which turns the target off. The intended method for turning a target off is to set Target_State=0. <BR>
      | <P>
      | <B>Opacity:</B> This input is only available if Source for Opacity is selected as port, in which case the opacity for all of the targets created by this block is specified as a percentage.
      | The length of this input must either match the length of the Target_Row(s) input (i.e. which case each Opacity maps to the appropriate Target_row)
      | or this input must be a scalar (in which case the Opacity maps to all of the Target_Rows).<BR>
      | <P>
      | There is one output from this block:
      | <P>
      | <B> VCODE: </B> this output is a vector containing one VCODE. This output must go to the Process_Video_CMD block of the video library for the target to actually be shown (if any other visual targets are to be displayed, then this VCODE output must be concatenated with the other VCODES prior to connection to the Process_Video_CMD block - see Help for the Process_Video_CMD block for more information).
      | <P>
      | To show multiple targets simultaneously, multiple copies of the Show_Target and Show_Target_With_Label blocks can be used in a Task Program. The output VCODES from multiple Show_Target and Show_Target_With_Label blocks must be concatenated prior to connection to the Process_Video_CMD block.
      | <P>
      | 
      | <H2>Parameters and Dialog Box</H2>
      | <B>Type of Target:</B> Choose the type of target specified in the target table.
      | <P>
      | <B>Number of Target States:</B> Choose the number of target states specified in each target row. Up to five target states are allowed per target row.
      | <P>
      | <B>State [n] Target Table Columns:</B> Enter the column indices that specify the relevant target attributes in the Target Table. All target types have the same first three target attributes (fill colour, stroke colour and stroke width) and the same last three target attributes (label text, label colour, and label height).
      | <Blockquote>
      | <P>
      | Element 1 (fill colour) - points to the column index in the Target Table containing the fill colour. If this index is 0, then the fill colour is transparent and the Target Table is not referenced. For line targets, the fill colour is not used.
      | <P>
      | Element 2 (stroke colour) - points to the column index in the Target Table containing the stroke colour. If this index is 0, then the stroke colour is transparent and the Target Table is not referenced. It is possible to use the same column index for both fill colour and stroke colour (i.e.  if single-colour targets are desired). For line targets, stroke colour defines the colour of the line.
      | <P>
      | Element 3 (stroke width) - points to the column index in the Target Table containing the stroke width (cm). If no stroke is desired, then setting the stroke column index to 0 will produce a stroke width of 0  and the Target Table is not referenced.  Setting stroke column index to a value less than 0 will produce a standard 1 mm stroke width, again without referencing the Target Table. For line targets, stroke width defines the width of the line.
      | <P>
      | <B><I>Circle</I></B> <P>
      | Element 4 (radius) - radius of the circle (cm).
      | <P>
      | <B><I>Ellipse</I></B> <P>
      | Elements 4-6 (ellipse properties) - major radius (cm), minor radius (cm), rotation angle (degrees). If no rotation is desired, then setting rotation column index to 0 will produce a default rotation of 0 and the Target Table will not be referenced.
      | <P>
      | <B><I>Rectangle</I></B><P>
      | Elements 4-6 (rectangle properties) - length (cm), height (cm), rotation angle (degrees). If no rotation is desired, then setting rotation column index to 0 will produce a default rotation of 0 and the Target Table will not be referenced.
      | <P>
      | <B><I>Line</I></B><P>
      | Elements 4-5 (line properties) - end point x-axis position relative to start point (cm), end point y-axis position relative to start point (cm). The width and colour of the line are defined by the stroke width and the stroke colour, respectively. The fill colour column is ignored (i.e. any value can be used for column 1)
      | <P>
      | <B><I>Triangle</I></B><P>
      | Elements 4-7 (triangle properties) - length (cm), height (cm), offset of peak of triangle relative to midpoint of the length (cm), rotation angle (degrees). If a height column index of 0 is specified, then an equilateral triangle with sides of the specified length will be created and the Target Table will not be referenced for height or peak offset. If no rotation is desired, then setting a rotation column index of 0 will produce a default rotation of 0 and the Target Table will not be referenced.
      | <P>
      | <B><I>Label</I></B>
      | <P>
      | The last three elements of the target state vector define the label. In order, these elements are:
      | <P>
      | Label text - the index of the column in the Target Table containing the text used for the label (up to 50 characters).
      | <P>
      | Label colour - the index of the column in the Target Table containing the label colour. If this index is 0, then the label colour is transparent and the Target Table is not referenced.
      | <P>
      | Label height - the index of the column in the Target Table containing the label height (cm).
      | </Blockquote>
      | <P>
      | Each target state requires its own set of column index definitions (although multiple states can point to the same column index if desired).<P>
      | 
      | <B>Source for Opacity:</B> Choose either dialog, to specify the opacity in this dialog, or port, which will create a new input to allow dynamic control of opacity.
      | <P>
      | <B>Opacity:</B> This parameter is only available if Source for Opacity is selected as dialog, in which case the opacity for all of the targets created by this block is specified as a percentage.
      | <P>
      | <B>Target Display:</B> This option determines whether the target(s) are shown on the operator display only, the subject display only, or both displays.
      | <P>
      | 
      | <H2>Examples</H2>
      | 
      | <B>Example 1:</B>  Suppose a target row will be used to define 1 state for an ellipse type target. It will be an outline of an ellipse with a label in the center (using a stroke colour and a standard 1mm stroke width). The related Target Table columns are:
      | <P>
      | column 4 = colour<BR>
      | column 5 = major radius<BR>
      | column 6 = minor radius<BR>
      | column 7 = orientation<BR>
      | column 8 = label text<BR>
      | column 9 = label colour<BR>
      | column 10 = label height
      | <P>For this example, "State 1 Target Table Columns" would equal [0 4 -1 5 6 7 8 9 10].
      | <P>
      | 
      | <H2>Related Blocks </H2>
      | Show_Target<BR>
      | Process_Video_CMD
      mask TypeOptions target_type: Circle | Ellipse | Rectangle | Line | Triangle
      mask Callback target_type:
      | %%%%
      | % Because of bugs iN R2007, R2010a and R2013a (which have been reported to Mathworks), the following code
      | % is required here because in the Initialization Section it will ONLY correctly update those Mask Parameters that are hidden
      | % when the OK button is clicked (NOTE: the initialization code will correctly update all Mask Parameters when the Apply button
      | % is clicked, the bug is that it should also update everything when the OK button is clicked in the absence of an Apply click)
      | %
      | % Adding a set_param call which updates one of the mask parameters will call the initialization code to run, which "avoids"
      | % this bug. This code should be removed once Mathworks has fixed this bug.
      | 
      | temp = get_param(gcb, 'target_type');
      | set_param(gcb, 'target_type', temp);
      mask TypeOptions num_states: 1 | 2 | 3 | 4 | 5
      mask Callback num_states:
      | block_path=gcb;
      | num_states=str2num(get_param(block_path, 'num_states'));
      | vis=get_param(block_path,'MaskVisibilities');
      | 
      | %If the number of states>1, then output an array instead of a vector.
      | %Only show those inputs necessary on the Mask
      | output_block=char(find_system(block_path,'LookUnderMasks','all','SearchDepth',1,'BlockType','Outport'));
      | if num_states==1			%output of HandInTarget block is a vector
      | 	vis{4}='off';
      | 	vis{5}='off';
      | 	vis{6}='off';
      | 	vis{7}='off';
      | elseif num_states==2					%output of HandInTarget block is an array
      | 	vis{4}='on';
      | 	vis{5}='off';
      | 	vis{6}='off';
      | 	vis{7}='off';
      | elseif num_states==3					%output of HandInTarget block is an array
      | 	vis{4}='on';
      | 	vis{5}='on';
      | 	vis{6}='off';
      | 	vis{7}='off';
      | elseif num_states==4					%output of HandInTarget block is an array
      | 	vis{4}='on';
      | 	vis{5}='on';
      | 	vis{6}='on';
      | 	vis{7}='off';
      | else								%output of HandInTarget block is an array
      | 	vis{4}='on';
      | 	vis{5}='on';
      | 	vis{6}='on';
      | 	vis{7}='on';
      | end
      | set_param(block_path,'MaskVisibilities',vis);
      mask TypeOptions source: dialog | port
      mask Callback source:
      | % Show or hide the opacity input on the mask dialog
      | sourceStr=get_param(gcb,'source');
      | vis=get_param(gcb,'MaskVisibilities');
      | 
      | if strmatch(sourceStr, 'dialog')
      | 	vis{10}='on';
      | else
      | 	vis{10}='off';
      | end
      | 
      | set_param(gcb,'MaskVisibilities',vis);
      mask TypeOptions target_display: Both subject and operator displays | Subject display only | Operator display only
      mask Display: disp(columntext); port_label('output',1,outputname); port_label('input',1, inputname1); port_label('input',2, inputname2);
  Process_Video_CMD : Video/Process_Video_CMD
  Scope (xPC) 2 : xpclib/Misc./Scope (xPC)   Priority=1  scopeno=2  scopetype=Target  autostart=on  viewmode=Numerical  formatstr='%15.6f'  grid=on  ylimits=[-0.3,0.3]  nosamples=1000  noprepostsamples=0  interleave=5  triggermode=FreeRun  triggersignal=1  trigsignalfromport=off  triggerlevel=0.0  triggerslope=Either  triggerscope=1  triggersample=0  filename=data.dat  mode=Lazy  writesize=512  autorestart=off  dynamicfilemode=off  maxwritefilesize=512*1024^2
  Selector1 : Selector  NumberOfDimensions=2  InputPortWidth=3  IndexOptions=Select all,Starting index (port)  Indices=[1 3],1  OutputSizes=1,1
  Selector17 : Selector  NumberOfDimensions=2  InputPortWidth=1  IndexOptions=Select all,Starting index (port)  Indices=[1 3],1  OutputSizes=1,1
  Selector2 : Selector  NumberOfDimensions=2  InputPortWidth=3  IndexOptions=Index vector (port),Select all  Indices=[1 3],1  OutputSizes=1,1
  Selector5 : Selector  NumberOfDimensions=2  InputPortWidth=3  IndexOptions=Select all,Starting index (port)  Indices=[1 3],1  OutputSizes=1,1
  Trajectory subsystem : Subsystem
  Trial_Control : Stateflow chart  TreatAsAtomicUnit=on
  function : MATLAB Function  TreatAsAtomicUnit=on
  Constant : Constant  IOType=siggen
  tag scope: CursorOpacity=global, ForceOn=global, HandVelX=global, HandVelY=global, OpacityGradient=global, trial_state=global, xEnd=global, xStart=global, yEnd=global, yStart=global
  wires:
  GUI Control/1 -> Trial_Control/Trigger
  Trial_Control/1(logging_enable) -> DataLogging/1
  Trial_Control/5(e_Trial_End) -> GUI Control/1
  Trajectory subsystem/2(EXO Torques) -> KINARM_Apply_Loads/1
  Trajectory subsystem/1(EP forces) -> KINARM_EP_Apply_Loads/1
  Constant4/1 -> Parameter_columns/2(Target_State)
  Parameter_columns/1(VCODE) -> Hand_at_start/1(SET_EXP_PARAMS1)
  Draw_Hand_Endpoint/1(VCODE) -> Trajectory subsystem/2(target_position), Matrix Concatenate/1
  [KINdata] -> Hand_at_start/2(KINdata)
  Hand_at_start/1(HandAtStart) -> Trial_Control/2(HandAtStart)
  Trial_Control/2(trial_state) -> Mux2/1, [trial_state], Mux/1
  Mux/1 -> DataLogging/2
  Constant1/1 -> Draw_End_Circle/2(Target_State), Draw_End_Circle/1(Target_Row), Draw_Start_Circle/2(Target_State), Draw_Start_Circle/1(Target_Row), Draw_Hand_Endpoint/1(Target_Row), Draw_Hand_Endpoint/2(Target_State)
  Matrix Concatenate/1 -> Process_Video_CMD/1
  Trial_Control/3(ForceOn) -> [ForceOn]
  Constant5/1 -> Selector1/2
  Selector1/1 -> Parameter_columns/1(Target_Row)
  Constant6/1 -> Trajectory subsystem/1(Duration)
  Draw_Start_Circle/1(VCODE) -> Matrix Concatenate/2
  Selector5/1 -> Selector2/2
  [Load_Table] -> Selector2/1
  Selector2/1 -> Selector17/1
  Mux2/1 -> Scope (xPC) 2/1
  Hand_at_start/2(xStart) -> [xStart]
  Hand_at_start/3(yStart) -> [yStart]
  Draw_End_Circle/1(VCODE) -> Matrix Concatenate/3
  Hand_at_start/4(xEnd) -> [xEnd]
  Hand_at_start/5(yEnd) -> [yEnd]
  Hand_at_start/6(HandVelX) -> [HandVelX]
  Hand_at_start/7(HandVelY) -> [HandVelY]
  [HandVelX] -> Mux/2
  [HandVelY] -> Mux/3
  [trial_state] -> function/1(trial_state)
  Constant2/1 -> Selector17/2
  Selector17/1 -> [OpacityGradient]
  [OpacityGradient] -> function/2(OpacityGradient)
  function/1(CursorOpacity) -> Mux2/2, [CursorOpacity]
  function/2(TrialTimeOut) -> Mux2/3
  GUI Control/2 -> Trial_Control/1(Trial_Protocol), Selector5/1, Selector1/1
  Constant3/1 -> Selector5/2
